simulink model "tb_speed_control"  (R2025b)
settings: Solver=VariableStepAuto  StopTime=0.2  FixedStep=control.currentLoopPeriod_s  MaxStep=1e-5  RelTol=1e-6  AbsTol=1e-9
undefined symbols (not defined in the file or in its folder): control, speedControl
settings Model: Creator=semih  LastModifiedBy=Semih
settings SFSimCC: SimGPUStackLimitPerThread=51200  SimGPUMallocThreshold=200
settings RTWCC: GPUStackLimitPerThread=51200  GPUMallocThreshold=200

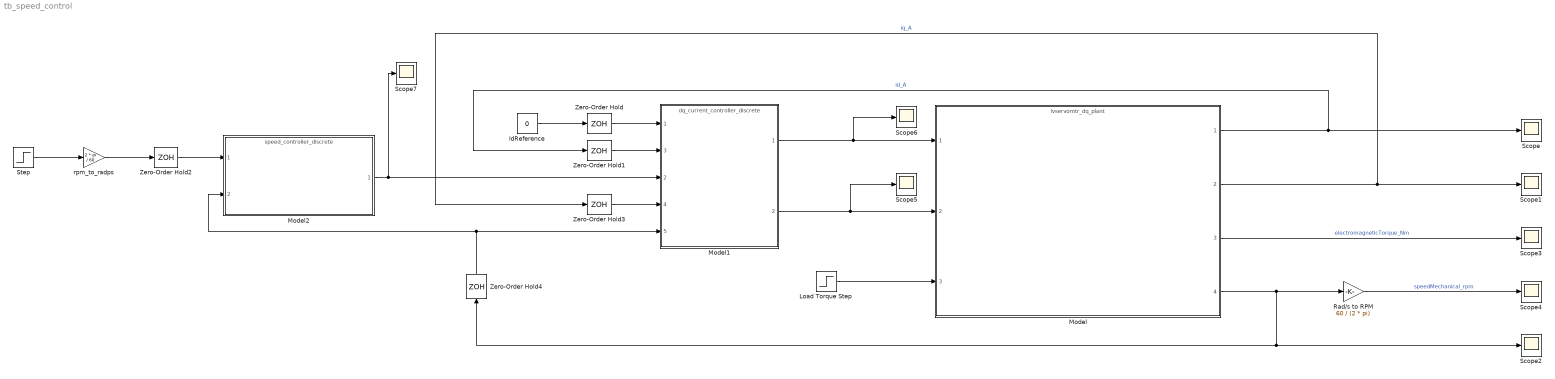
== system tb_speed_control ==
  IdReference : Constant  Value=0
  Load Torque Step : Step  Time=0.04  After=0.02  SampleTime=0
  Model : ModelReference  ModelNameDialog=lvservomtr_dq_plant  SimulationMode=Normal  ModelReferenceVersion=1.8
  Model1 : ModelReference  ModelNameDialog=dq_current_controller_discrete.slx  SimulationMode=Normal  ModelReferenceVersion=3.19
      settings: PortSchema="{\"entries\":[{\"content\":{\"sides\":[{\"content\":{\"connectorIds\":[\"In1\",\"In3\",\"In2\",\"In4\",\"In5\"]},\"type\":\"ConnectorPlacement.EquallySpacedRectSide\",\"uuid\":\"770debb9-2b2b-46a4-b6d4-b3cc8bc40512\"},{\"content\":{\"connectorIds\":[\"Out1\",\"Out2\"],\"side\":\"RIGHT\"},\"type\":\"ConnectorPlacement.EquallySpacedRectSide\",\"uuid\":\"10529b08-f942-4ed5-be6b-2ca61e24ccbd\"},{\"content\":{\"side\":\"TOP\"},\"type\":\"ConnectorPlacement.EquallySpacedRectSide\",\"uuid\":\"f8c183bf-1389-4593-9ed4-5d7ce061c30e\"}]},\"type\":\"ConnectorPlacement.EquallySpacedConnector\",\"uuid\":\"7720b2ba-7d08-46f0-a5d3-6c147234f35e\"}],\"packageUris\":[\"http://schema.mathworks.com/mf0/Connector/R2020b\"],\"version\":\"1.0\"}"
  Model2 : ModelReference  ModelNameDialog=speed_controller_discrete.slx  SimulationMode=Normal  ModelReferenceVersion=1.0
  Rad/s to RPM : Gain  Gain=60 / (2 * pi)
  Scope{,1..7} (8 alike) : Scope
      Scope settings: ActiveDisplayYMinimum=-6.4319807901886685E-5  ActiveDisplayYMaximum=0.00063213654626412632
      Scope1 settings: ActiveDisplayYMinimum=-0.42519345981876139  ActiveDisplayYMaximum=2.9261140651176016
      Scope2 settings: ActiveDisplayYMinimum=5.6456577172899642  ActiveDisplayYMaximum=93.825222343411241  DataLoggingVariableName=ScopeData2
      Scope3 settings: ActiveDisplayYMinimum=-0.060906186129986689  ActiveDisplayYMaximum=0.13304762379593027  DataLoggingVariableName=ScopeData3
      Scope4 settings: ActiveDisplayYMinimum=-18.323398026151015  ActiveDisplayYMaximum=206.42801209105286  DataLoggingVariableName=ScopeData4
      Scope5 settings: ActiveDisplayYMinimum=-0.8660254037844386  ActiveDisplayYMaximum=7.79422863405995  DataLoggingVariableName=ScopeData5
      Scope6 settings: ActiveDisplayYMinimum=-0.68910289578742845  ActiveDisplayYMaximum=0.14221325534308124  DataLoggingVariableName=ScopeData6
      Scope7 settings: ActiveDisplayYMinimum=-0.12917896613505417  ActiveDisplayYMaximum=1.4589277691225249  DataLoggingVariableName=ScopeData7
  Step : Step  Time=0.005  After=100  SampleTime=0
  Zero-Order Hold{,1,3..4} (4 alike) : ZeroOrderHold  SampleTime=control.currentLoopPeriod_s
  Zero-Order Hold2 : ZeroOrderHold  SampleTime=speedControl.sampleTime_s
  rpm_to_radps : Gain  Gain=2 * pi / 60
  wires:
  Load Torque Step/1 -> Model/3
  Rad/s to RPM/1 -> Scope4/1  "speedMechanical_rpm"
  Model/4 -> Zero-Order Hold4/1, Scope2/1, Rad/s to RPM/1
  Model1/2 -> Scope5/1, Model/2
  Model/3 -> Scope3/1  "electromagneticTorque_Nm"
  Model/1 -> Zero-Order Hold1/1, Scope/1  "id_A"
  Model/2 -> Zero-Order Hold3/1, Scope1/1  "iq_A"
  Model1/1 -> Scope6/1, Model/1
  IdReference/1 -> Zero-Order Hold/1
  Zero-Order Hold/1 -> Model1/1
  Zero-Order Hold1/1 -> Model1/3
  Zero-Order Hold3/1 -> Model1/4
  Step/1 -> rpm_to_radps/1
  rpm_to_radps/1 -> Zero-Order Hold2/1
  Zero-Order Hold2/1 -> Model2/1
  Model2/1 -> Scope7/1, Model1/2
  Zero-Order Hold4/1 -> Model1/5, Model2/2
